simulink model "r23_512p_fft"  (R2026b)
settings: Solver=FixedStepDiscrete  StopTime=5e-5*(127-1)  FixedStep=5e-5
libraries: dspsrcs4 x8
(part 2 of 3)

== matlab function r23_512p_fft/FFT_TOP/calc_unit29/r2_unit ==
  data: si_cha input; so_cha output; so_chb output; si_chb input
function [so_cha, so_chb] = r2_unit(si_cha, si_chb)
%R2_UNIT Radix-2 butterfly.

DW = 15;
fm = fimath('RoundingMethod', 'Nearest', 'OverflowAction', 'Saturate', ...
    'ProductMode', 'FullPrecision', 'SumMode', 'FullPrecision');

so_cha = fi(zeros(1, 2), 1, DW, 0, fm);
so_chb = fi(zeros(1, 2), 1, DW, 0, fm);
so_cha(:) = si_cha + si_chb;
so_chb(:) = si_cha - si_chb;
end

== matlab function r23_512p_fft/FFT_TOP/calc_unit34/r2_unit ==
  data: si_cha input; so_cha output; so_chb output; si_chb input
function [so_cha, so_chb] = r2_unit(si_cha, si_chb)
%R2_UNIT Radix-2 butterfly.

DW = 16;
fm = fimath('RoundingMethod', 'Nearest', 'OverflowAction', 'Saturate', ...
    'ProductMode', 'FullPrecision', 'SumMode', 'FullPrecision');

so_cha = fi(zeros(1, 2), 1, DW, 0, fm);
so_chb = fi(zeros(1, 2), 1, DW, 0, fm);
so_cha(:) = si_cha + si_chb;
so_chb(:) = si_cha - si_chb;
end

== matlab function r23_512p_fft/FFT_TOP/calc_unit17/pwr_unit ==
  data: si_cha input; so_cha output; so_chb output; si_chb input
function [so_cha, so_chb] = pwr_unit(si_cha, si_chb)
%PWR_UNIT Twiddle multiply before the butterfly: W^0, W^128.

DW = 13;
fm = fimath('RoundingMethod', 'Nearest', 'OverflowAction', 'Saturate', ...
    'ProductMode', 'FullPrecision', 'SumMode', 'FullPrecision');

so_cha = mul_one(si_cha, DW, fm);
so_chb = mul_neg_j(si_chb, DW, fm);
end

function y = mul_one(x, DW, fm)
y = fi(zeros(1, 2), 1, DW, 0, fm);
y(:) = x;
end

function y = mul_neg_j(x, DW, fm)
y = fi(zeros(1, 2), 1, DW, 0, fm);
y(1) = x(2);
y(2) = -x(1);
end

== matlab function r23_512p_fft/FFT_TOP/calc_unit35/r2_unit ==
  data: si_cha input; so_cha output; so_chb output; si_chb input
function [so_cha, so_chb] = r2_unit(si_cha, si_chb)
%R2_UNIT Radix-2 butterfly.

DW = 16;
fm = fimath('RoundingMethod', 'Nearest', 'OverflowAction', 'Saturate', ...
    'ProductMode', 'FullPrecision', 'SumMode', 'FullPrecision');

so_cha = fi(zeros(1, 2), 1, DW, 0, fm);
so_chb = fi(zeros(1, 2), 1, DW, 0, fm);
so_cha(:) = si_cha + si_chb;
so_chb(:) = si_cha - si_chb;
end

== matlab function r23_512p_fft/FFT_TOP/calc_unit32/r2_unit ==
  data: si_cha input; so_cha output; so_chb output; si_chb input
function [so_cha, so_chb] = r2_unit(si_cha, si_chb)
%R2_UNIT Radix-2 butterfly.

DW = 16;
fm = fimath('RoundingMethod', 'Nearest', 'OverflowAction', 'Saturate', ...
    'ProductMode', 'FullPrecision', 'SumMode', 'FullPrecision');

so_cha = fi(zeros(1, 2), 1, DW, 0, fm);
so_chb = fi(zeros(1, 2), 1, DW, 0, fm);
so_cha(:) = si_cha + si_chb;
so_chb(:) = si_cha - si_chb;
end

== matlab function r23_512p_fft/FFT_TOP/calc_unit0/r2_unit ==
  data: si_cha input; so_cha output; so_chb output; si_chb input
function [so_cha, so_chb] = r2_unit(si_cha, si_chb)
%R2_UNIT Radix-2 butterfly.

DW = 12;
fm = fimath('RoundingMethod', 'Nearest', 'OverflowAction', 'Saturate', ...
    'ProductMode', 'FullPrecision', 'SumMode', 'FullPrecision');

so_cha = fi(zeros(1, 2), 1, DW, 0, fm);
so_chb = fi(zeros(1, 2), 1, DW, 0, fm);
so_cha(:) = si_cha + si_chb;
so_chb(:) = si_cha - si_chb;
end

== matlab function r23_512p_fft/FFT_TOP/calc_unit33/r2_unit ==
  data: si_cha input; so_cha output; so_chb output; si_chb input
function [so_cha, so_chb] = r2_unit(si_cha, si_chb)
%R2_UNIT Radix-2 butterfly.

DW = 16;
fm = fimath('RoundingMethod', 'Nearest', 'OverflowAction', 'Saturate', ...
    'ProductMode', 'FullPrecision', 'SumMode', 'FullPrecision');

so_cha = fi(zeros(1, 2), 1, DW, 0, fm);
so_chb = fi(zeros(1, 2), 1, DW, 0, fm);
so_cha(:) = si_cha + si_chb;
so_chb(:) = si_cha - si_chb;
end

== matlab function r23_512p_fft/FFT_TOP/comm_unit01/sw_unit ==
  data: si_cha input; so_cha output; so_chb output; si_chb input
function [so_cha, so_chb] = sw_unit(si_cha, si_chb)
%SW_UNIT Commutator switch, depth 32.

N  = 32;
CW = 5;
DW = 12;
fm = fimath('RoundingMethod', 'Nearest', 'OverflowAction', 'Saturate', ...
    'ProductMode', 'FullPrecision', 'SumMode', 'FullPrecision');
fc = fimath('RoundingMethod', 'Floor', 'OverflowAction', 'Wrap', ...
    'ProductMode', 'FullPrecision', 'SumMode', 'FullPrecision');

persistent cnt sel
if isempty(cnt)
    cnt = fi(N - 1, 0, CW, 0, fc);
end
if isempty(sel)
    sel = true;
end

if cnt == N - 1
    cnt(:) = 0;
else
    cnt(:) = cnt + 1;
end
if cnt == 0
    sel = ~sel;
end

so_cha = fi(zeros(1, 2), 1, DW, 0, fm);
so_chb = fi(zeros(1, 2), 1, DW, 0, fm);
if sel
    so_cha(:) = si_chb;
    so_chb(:) = si_cha;
else
    so_cha(:) = si_cha;
    so_chb(:) = si_chb;
end
end

== matlab function r23_512p_fft/FFT_TOP/comm_unit02/sw_unit ==
  data: si_cha input; so_cha output; so_chb output; si_chb input
function [so_cha, so_chb] = sw_unit(si_cha, si_chb)
%SW_UNIT Commutator switch, depth 32.

N  = 32;
CW = 5;
DW = 12;
fm = fimath('RoundingMethod', 'Nearest', 'OverflowAction', 'Saturate', ...
    'ProductMode', 'FullPrecision', 'SumMode', 'FullPrecision');
fc = fimath('RoundingMethod', 'Floor', 'OverflowAction', 'Wrap', ...
    'ProductMode', 'FullPrecision', 'SumMode', 'FullPrecision');

persistent cnt sel
if isempty(cnt)
    cnt = fi(N - 1, 0, CW, 0, fc);
end
if isempty(sel)
    sel = true;
end

if cnt == N - 1
    cnt(:) = 0;
else
    cnt(:) = cnt + 1;
end
if cnt == 0
    sel = ~sel;
end

so_cha = fi(zeros(1, 2), 1, DW, 0, fm);
so_chb = fi(zeros(1, 2), 1, DW, 0, fm);
if sel
    so_cha(:) = si_chb;
    so_chb(:) = si_cha;
else
    so_cha(:) = si_cha;
    so_chb(:) = si_chb;
end
end

== matlab function r23_512p_fft/FFT_TOP/calc_unit19/pwr_unit ==
  data: si_cha input; so_cha output; so_chb output; si_chb input
function [so_cha, so_chb] = pwr_unit(si_cha, si_chb)
%PWR_UNIT Twiddle multiply before the butterfly: W^0, W^128.

DW = 13;
fm = fimath('RoundingMethod', 'Nearest', 'OverflowAction', 'Saturate', ...
    'ProductMode', 'FullPrecision', 'SumMode', 'FullPrecision');

so_cha = mul_one(si_cha, DW, fm);
so_chb = mul_neg_j(si_chb, DW, fm);
end

function y = mul_one(x, DW, fm)
y = fi(zeros(1, 2), 1, DW, 0, fm);
y(:) = x;
end

function y = mul_neg_j(x, DW, fm)
y = fi(zeros(1, 2), 1, DW, 0, fm);
y(1) = x(2);
y(2) = -x(1);
end

== matlab function r23_512p_fft/FFT_TOP/comm_unit03/sw_unit ==
  data: si_cha input; so_cha output; so_chb output; si_chb input
function [so_cha, so_chb] = sw_unit(si_cha, si_chb)
%SW_UNIT Commutator switch, depth 32.

N  = 32;
CW = 5;
DW = 12;
fm = fimath('RoundingMethod', 'Nearest', 'OverflowAction', 'Saturate', ...
    'ProductMode', 'FullPrecision', 'SumMode', 'FullPrecision');
fc = fimath('RoundingMethod', 'Floor', 'OverflowAction', 'Wrap', ...
    'ProductMode', 'FullPrecision', 'SumMode', 'FullPrecision');

persistent cnt sel
if isempty(cnt)
    cnt = fi(N - 1, 0, CW, 0, fc);
end
if isempty(sel)
    sel = true;
end

if cnt == N - 1
    cnt(:) = 0;
else
    cnt(:) = cnt + 1;
end
if cnt == 0
    sel = ~sel;
end

so_cha = fi(zeros(1, 2), 1, DW, 0, fm);
so_chb = fi(zeros(1, 2), 1, DW, 0, fm);
if sel
    so_cha(:) = si_chb;
    so_chb(:) = si_cha;
else
    so_cha(:) = si_cha;
    so_chb(:) = si_chb;
end
end

== matlab function r23_512p_fft/FFT_TOP/comm_unit10/sw_unit ==
  data: si_cha input; so_cha output; so_chb output; si_chb input
function [so_cha, so_chb] = sw_unit(si_cha, si_chb)
%SW_UNIT Commutator switch, depth 16.

N  = 16;
CW = 4;
DW = 13;
fm = fimath('RoundingMethod', 'Nearest', 'OverflowAction', 'Saturate', ...
    'ProductMode', 'FullPrecision', 'SumMode', 'FullPrecision');
fc = fimath('RoundingMethod', 'Floor', 'OverflowAction', 'Wrap', ...
    'ProductMode', 'FullPrecision', 'SumMode', 'FullPrecision');

persistent cnt sel
if isempty(cnt)
    cnt = fi(N - 1, 0, CW, 0, fc);
end
if isempty(sel)
    sel = true;
end

if cnt == N - 1
    cnt(:) = 0;
else
    cnt(:) = cnt + 1;
end
if cnt == 0
    sel = ~sel;
end

so_cha = fi(zeros(1, 2), 1, DW, 0, fm);
so_chb = fi(zeros(1, 2), 1, DW, 0, fm);
if sel
    so_cha(:) = si_chb;
    so_chb(:) = si_cha;
else
    so_cha(:) = si_cha;
    so_chb(:) = si_chb;
end
end

== matlab function r23_512p_fft/FFT_TOP/comm_unit11/sw_unit ==
  data: si_cha input; so_cha output; so_chb output; si_chb input
function [so_cha, so_chb] = sw_unit(si_cha, si_chb)
%SW_UNIT Commutator switch, depth 16.

N  = 16;
CW = 4;
DW = 13;
fm = fimath('RoundingMethod', 'Nearest', 'OverflowAction', 'Saturate', ...
    'ProductMode', 'FullPrecision', 'SumMode', 'FullPrecision');
fc = fimath('RoundingMethod', 'Floor', 'OverflowAction', 'Wrap', ...
    'ProductMode', 'FullPrecision', 'SumMode', 'FullPrecision');

persistent cnt sel
if isempty(cnt)
    cnt = fi(N - 1, 0, CW, 0, fc);
end
if isempty(sel)
    sel = true;
end

if cnt == N - 1
    cnt(:) = 0;
else
    cnt(:) = cnt + 1;
end
if cnt == 0
    sel = ~sel;
end

so_cha = fi(zeros(1, 2), 1, DW, 0, fm);
so_chb = fi(zeros(1, 2), 1, DW, 0, fm);
if sel
    so_cha(:) = si_chb;
    so_chb(:) = si_cha;
else
    so_cha(:) = si_cha;
    so_chb(:) = si_chb;
end
end

== matlab function r23_512p_fft/FFT_TOP/calc_unit2/r2_unit ==
  data: si_cha input; so_cha output; so_chb output; si_chb input
function [so_cha, so_chb] = r2_unit(si_cha, si_chb)
%R2_UNIT Radix-2 butterfly.

DW = 12;
fm = fimath('RoundingMethod', 'Nearest', 'OverflowAction', 'Saturate', ...
    'ProductMode', 'FullPrecision', 'SumMode', 'FullPrecision');

so_cha = fi(zeros(1, 2), 1, DW, 0, fm);
so_chb = fi(zeros(1, 2), 1, DW, 0, fm);
so_cha(:) = si_cha + si_chb;
so_chb(:) = si_cha - si_chb;
end

== matlab function r23_512p_fft/FFT_TOP/calc_unit20/bwr_unit ==
  data: si_cha input; so_cha output; so_chb output; si_chb input
function [so_cha, so_chb] = bwr_unit(si_cha, si_chb)
%BWR_UNIT Twiddle multiply after the butterfly: W^(8k), W^(40k), k = 0..7.

DW = 15;
LEN = 8;
KW  = 3;
fm = fimath('RoundingMethod', 'Nearest', 'OverflowAction', 'Saturate', ...
    'ProductMode', 'FullPrecision', 'SumMode', 'FullPrecision');
fc = fimath('RoundingMethod', 'Floor', 'OverflowAction', 'Wrap', ...
    'ProductMode', 'FullPrecision', 'SumMode', 'FullPrecision');
ROM_A_RE = coder.const(twiddle((0:LEN-1).' * 8, 1, fm));
ROM_A_IM = coder.const(twiddle((0:LEN-1).' * 8, 2, fm));
ROM_B_RE = coder.const(twiddle((0:LEN-1).' * 40, 1, fm));
ROM_B_IM = coder.const(twiddle((0:LEN-1).' * 40, 2, fm));

persistent k
if isempty(k)
    k = fi(LEN - 1, 0, KW, 0, fc);
end
if k == LEN - 1
    k(:) = 0;
else
    k(:) = k + 1;
end

so_cha = cmul(si_cha, [ROM_A_RE(k + 1), ROM_A_IM(k + 1)], DW, fm);
so_chb = cmul(si_chb, [ROM_B_RE(k + 1), ROM_B_IM(k + 1)], DW, fm);
end

function y = cmul(x, w, DW, fm)
y = fi(zeros(1, 2), 1, DW, 0, fm);
y(1) = x(1)*w(1) - x(2)*w(2);
y(2) = x(2)*w(1) + x(1)*w(2);
end

function w = twiddle(k, part, fm)
if part == 1
    w = fi(cos(2*pi*k/512), 1, 10, 8, fm);
else
    w = fi(-sin(2*pi*k/512), 1, 10, 8, fm);
end
end

== matlab function r23_512p_fft/FFT_TOP/calc_unit20/pwr_unit ==
  data: si_cha input; so_cha output; so_chb output; si_chb input
function [so_cha, so_chb] = pwr_unit(si_cha, si_chb)
%PWR_UNIT Twiddle multiply before the butterfly: W^0, W^64.

DW = 14;
fm = fimath('RoundingMethod', 'Nearest', 'OverflowAction', 'Saturate', ...
    'ProductMode', 'FullPrecision', 'SumMode', 'FullPrecision');
W_B = coder.const([twiddle(64, 1, fm), twiddle(64, 2, fm)]);

so_cha = mul_one(si_cha, DW, fm);
so_chb = cmul(si_chb, W_B, DW, fm);
end

function y = mul_one(x, DW, fm)
y = fi(zeros(1, 2), 1, DW, 0, fm);
y(:) = x;
end

function y = cmul(x, w, DW, fm)
y = fi(zeros(1, 2), 1, DW, 0, fm);
y(1) = x(1)*w(1) - x(2)*w(2);
y(2) = x(2)*w(1) + x(1)*w(2);
end

function w = twiddle(k, part, fm)
if part == 1
    w = fi(cos(2*pi*k/512), 1, 10, 8, fm);
else
    w = fi(-sin(2*pi*k/512), 1, 10, 8, fm);
end
end

== matlab function r23_512p_fft/FFT_TOP/calc_unit1/bwr_unit ==
  data: si_cha input; so_cha output; so_chb output; si_chb input
function [so_cha, so_chb] = bwr_unit(si_cha, si_chb)
%BWR_UNIT Twiddle multiply after the butterfly: W^0, W^128.

DW = 12;
fm = fimath('RoundingMethod', 'Nearest', 'OverflowAction', 'Saturate', ...
    'ProductMode', 'FullPrecision', 'SumMode', 'FullPrecision');

so_cha = mul_one(si_cha, DW, fm);
so_chb = mul_neg_j(si_chb, DW, fm);
end

function y = mul_one(x, DW, fm)
y = fi(zeros(1, 2), 1, DW, 0, fm);
y(:) = x;
end

function y = mul_neg_j(x, DW, fm)
y = fi(zeros(1, 2), 1, DW, 0, fm);
y(1) = x(2);
y(2) = -x(1);
end

== matlab function r23_512p_fft/FFT_TOP/comm_unit12/sw_unit ==
  data: si_cha input; so_cha output; so_chb output; si_chb input
function [so_cha, so_chb] = sw_unit(si_cha, si_chb)
%SW_UNIT Commutator switch, depth 16.

N  = 16;
CW = 4;
DW = 13;
fm = fimath('RoundingMethod', 'Nearest', 'OverflowAction', 'Saturate', ...
    'ProductMode', 'FullPrecision', 'SumMode', 'FullPrecision');
fc = fimath('RoundingMethod', 'Floor', 'OverflowAction', 'Wrap', ...
    'ProductMode', 'FullPrecision', 'SumMode', 'FullPrecision');

persistent cnt sel
if isempty(cnt)
    cnt = fi(N - 1, 0, CW, 0, fc);
end
if isempty(sel)
    sel = true;
end

if cnt == N - 1
    cnt(:) = 0;
else
    cnt(:) = cnt + 1;
end
if cnt == 0
    sel = ~sel;
end

so_cha = fi(zeros(1, 2), 1, DW, 0, fm);
so_chb = fi(zeros(1, 2), 1, DW, 0, fm);
if sel
    so_cha(:) = si_chb;
    so_chb(:) = si_cha;
else
    so_cha(:) = si_cha;
    so_chb(:) = si_chb;
end
end

== matlab function r23_512p_fft/FFT_TOP/calc_unit21/bwr_unit ==
  data: si_cha input; so_cha output; so_chb output; si_chb input
function [so_cha, so_chb] = bwr_unit(si_cha, si_chb)
%BWR_UNIT Twiddle multiply after the butterfly: W^(24k), W^(56k), k = 0..7.

DW = 15;
LEN = 8;
KW  = 3;
fm = fimath('RoundingMethod', 'Nearest', 'OverflowAction', 'Saturate', ...
    'ProductMode', 'FullPrecision', 'SumMode', 'FullPrecision');
fc = fimath('RoundingMethod', 'Floor', 'OverflowAction', 'Wrap', ...
    'ProductMode', 'FullPrecision', 'SumMode', 'FullPrecision');
ROM_A_RE = coder.const(twiddle((0:LEN-1).' * 24, 1, fm));
ROM_A_IM = coder.const(twiddle((0:LEN-1).' * 24, 2, fm));
ROM_B_RE = coder.const(twiddle((0:LEN-1).' * 56, 1, fm));
ROM_B_IM = coder.const(twiddle((0:LEN-1).' * 56, 2, fm));

persistent k
if isempty(k)
    k = fi(LEN - 1, 0, KW, 0, fc);
end
if k == LEN - 1
    k(:) = 0;
else
    k(:) = k + 1;
end

so_cha = cmul(si_cha, [ROM_A_RE(k + 1), ROM_A_IM(k + 1)], DW, fm);
so_chb = cmul(si_chb, [ROM_B_RE(k + 1), ROM_B_IM(k + 1)], DW, fm);
end

function y = cmul(x, w, DW, fm)
y = fi(zeros(1, 2), 1, DW, 0, fm);
y(1) = x(1)*w(1) - x(2)*w(2);
y(2) = x(2)*w(1) + x(1)*w(2);
end

function w = twiddle(k, part, fm)
if part == 1
    w = fi(cos(2*pi*k/512), 1, 10, 8, fm);
else
    w = fi(-sin(2*pi*k/512), 1, 10, 8, fm);
end
end

== matlab function r23_512p_fft/FFT_TOP/calc_unit21/pwr_unit ==
  data: si_cha input; so_cha output; so_chb output; si_chb input
function [so_cha, so_chb] = pwr_unit(si_cha, si_chb)
%PWR_UNIT Twiddle multiply before the butterfly: W^0, W^192.

DW = 14;
fm = fimath('RoundingMethod', 'Nearest', 'OverflowAction', 'Saturate', ...
    'ProductMode', 'FullPrecision', 'SumMode', 'FullPrecision');
W_B = coder.const([twiddle(192, 1, fm), twiddle(192, 2, fm)]);

so_cha = mul_one(si_cha, DW, fm);
so_chb = cmul(si_chb, W_B, DW, fm);
end

function y = mul_one(x, DW, fm)
y = fi(zeros(1, 2), 1, DW, 0, fm);
y(:) = x;
end

function y = cmul(x, w, DW, fm)
y = fi(zeros(1, 2), 1, DW, 0, fm);
y(1) = x(1)*w(1) - x(2)*w(2);
y(2) = x(2)*w(1) + x(1)*w(2);
end

function w = twiddle(k, part, fm)
if part == 1
    w = fi(cos(2*pi*k/512), 1, 10, 8, fm);
else
    w = fi(-sin(2*pi*k/512), 1, 10, 8, fm);
end
end

== matlab function r23_512p_fft/FFT_TOP/comm_unit13/sw_unit ==
  data: si_cha input; so_cha output; so_chb output; si_chb input
function [so_cha, so_chb] = sw_unit(si_cha, si_chb)
%SW_UNIT Commutator switch, depth 16.

N  = 16;
CW = 4;
DW = 13;
fm = fimath('RoundingMethod', 'Nearest', 'OverflowAction', 'Saturate', ...
    'ProductMode', 'FullPrecision', 'SumMode', 'FullPrecision');
fc = fimath('RoundingMethod', 'Floor', 'OverflowAction', 'Wrap', ...
    'ProductMode', 'FullPrecision', 'SumMode', 'FullPrecision');

persistent cnt sel
if isempty(cnt)
    cnt = fi(N - 1, 0, CW, 0, fc);
end
if isempty(sel)
    sel = true;
end

if cnt == N - 1
    cnt(:) = 0;
else
    cnt(:) = cnt + 1;
end
if cnt == 0
    sel = ~sel;
end

so_cha = fi(zeros(1, 2), 1, DW, 0, fm);
so_chb = fi(zeros(1, 2), 1, DW, 0, fm);
if sel
    so_cha(:) = si_chb;
    so_chb(:) = si_cha;
else
    so_cha(:) = si_cha;
    so_chb(:) = si_chb;
end
end

== matlab function r23_512p_fft/FFT_TOP/calc_unit22/bwr_unit ==
  data: si_cha input; so_cha output; so_chb output; si_chb input
function [so_cha, so_chb] = bwr_unit(si_cha, si_chb)
%BWR_UNIT Twiddle multiply after the butterfly: W^0, W^(32k), k = 0..7.

DW = 15;
LEN = 8;
KW  = 3;
fm = fimath('RoundingMethod', 'Nearest', 'OverflowAction', 'Saturate', ...
    'ProductMode', 'FullPrecision', 'SumMode', 'FullPrecision');
fc = fimath('RoundingMethod', 'Floor', 'OverflowAction', 'Wrap', ...
    'ProductMode', 'FullPrecision', 'SumMode', 'FullPrecision');
ROM_B_RE = coder.const(twiddle((0:LEN-1).' * 32, 1, fm));
ROM_B_IM = coder.const(twiddle((0:LEN-1).' * 32, 2, fm));

persistent k
if isempty(k)
    k = fi(LEN - 1, 0, KW, 0, fc);
end
if k == LEN - 1
    k(:) = 0;
else
    k(:) = k + 1;
end

so_cha = mul_one(si_cha, DW, fm);
so_chb = cmul(si_chb, [ROM_B_RE(k + 1), ROM_B_IM(k + 1)], DW, fm);
end

function y = mul_one(x, DW, fm)
y = fi(zeros(1, 2), 1, DW, 0, fm);
y(:) = x;
end

function y = cmul(x, w, DW, fm)
y = fi(zeros(1, 2), 1, DW, 0, fm);
y(1) = x(1)*w(1) - x(2)*w(2);
y(2) = x(2)*w(1) + x(1)*w(2);
end

function w = twiddle(k, part, fm)
if part == 1
    w = fi(cos(2*pi*k/512), 1, 10, 8, fm);
else
    w = fi(-sin(2*pi*k/512), 1, 10, 8, fm);
end
end

== matlab function r23_512p_fft/FFT_TOP/comm_unit20/sw_unit ==
  data: si_cha input; so_cha output; so_chb output; si_chb input
function [so_cha, so_chb] = sw_unit(si_cha, si_chb)
%SW_UNIT Commutator switch, depth 8.

N  = 8;
CW = 3;
DW = 14;
fm = fimath('RoundingMethod', 'Nearest', 'OverflowAction', 'Saturate', ...
    'ProductMode', 'FullPrecision', 'SumMode', 'FullPrecision');
fc = fimath('RoundingMethod', 'Floor', 'OverflowAction', 'Wrap', ...
    'ProductMode', 'FullPrecision', 'SumMode', 'FullPrecision');

persistent cnt sel
if isempty(cnt)
    cnt = fi(N - 1, 0, CW, 0, fc);
end
if isempty(sel)
    sel = true;
end

if cnt == N - 1
    cnt(:) = 0;
else
    cnt(:) = cnt + 1;
end
if cnt == 0
    sel = ~sel;
end

so_cha = fi(zeros(1, 2), 1, DW, 0, fm);
so_chb = fi(zeros(1, 2), 1, DW, 0, fm);
if sel
    so_cha(:) = si_chb;
    so_chb(:) = si_cha;
else
    so_cha(:) = si_cha;
    so_chb(:) = si_chb;
end
end

== matlab function r23_512p_fft/FFT_TOP/comm_unit21/sw_unit ==
  data: si_cha input; so_cha output; so_chb output; si_chb input
function [so_cha, so_chb] = sw_unit(si_cha, si_chb)
%SW_UNIT Commutator switch, depth 8.

N  = 8;
CW = 3;
DW = 14;
fm = fimath('RoundingMethod', 'Nearest', 'OverflowAction', 'Saturate', ...
    'ProductMode', 'FullPrecision', 'SumMode', 'FullPrecision');
fc = fimath('RoundingMethod', 'Floor', 'OverflowAction', 'Wrap', ...
    'ProductMode', 'FullPrecision', 'SumMode', 'FullPrecision');

persistent cnt sel
if isempty(cnt)
    cnt = fi(N - 1, 0, CW, 0, fc);
end
if isempty(sel)
    sel = true;
end

if cnt == N - 1
    cnt(:) = 0;
else
    cnt(:) = cnt + 1;
end
if cnt == 0
    sel = ~sel;
end

so_cha = fi(zeros(1, 2), 1, DW, 0, fm);
so_chb = fi(zeros(1, 2), 1, DW, 0, fm);
if sel
    so_cha(:) = si_chb;
    so_chb(:) = si_cha;
else
    so_cha(:) = si_cha;
    so_chb(:) = si_chb;
end
end

== matlab function r23_512p_fft/FFT_TOP/calc_unit23/bwr_unit ==
  data: si_cha input; so_cha output; so_chb output; si_chb input
function [so_cha, so_chb] = bwr_unit(si_cha, si_chb)
%BWR_UNIT Twiddle multiply after the butterfly: W^(16k), W^(48k), k = 0..7.

DW = 15;
LEN = 8;
KW  = 3;
fm = fimath('RoundingMethod', 'Nearest', 'OverflowAction', 'Saturate', ...
    'ProductMode', 'FullPrecision', 'SumMode', 'FullPrecision');
fc = fimath('RoundingMethod', 'Floor', 'OverflowAction', 'Wrap', ...
    'ProductMode', 'FullPrecision', 'SumMode', 'FullPrecision');
ROM_A_RE = coder.const(twiddle((0:LEN-1).' * 16, 1, fm));
ROM_A_IM = coder.const(twiddle((0:LEN-1).' * 16, 2, fm));
ROM_B_RE = coder.const(twiddle((0:LEN-1).' * 48, 1, fm));
ROM_B_IM = coder.const(twiddle((0:LEN-1).' * 48, 2, fm));

persistent k
if isempty(k)
    k = fi(LEN - 1, 0, KW, 0, fc);
end
if k == LEN - 1
    k(:) = 0;
else
    k(:) = k + 1;
end

so_cha = cmul(si_cha, [ROM_A_RE(k + 1), ROM_A_IM(k + 1)], DW, fm);
so_chb = cmul(si_chb, [ROM_B_RE(k + 1), ROM_B_IM(k + 1)], DW, fm);
end

function y = cmul(x, w, DW, fm)
y = fi(zeros(1, 2), 1, DW, 0, fm);
y(1) = x(1)*w(1) - x(2)*w(2);
y(2) = x(2)*w(1) + x(1)*w(2);
end

function w = twiddle(k, part, fm)
if part == 1
    w = fi(cos(2*pi*k/512), 1, 10, 8, fm);
else
    w = fi(-sin(2*pi*k/512), 1, 10, 8, fm);
end
end

== matlab function r23_512p_fft/FFT_TOP/calc_unit23/pwr_unit ==
  data: si_cha input; so_cha output; so_chb output; si_chb input
function [so_cha, so_chb] = pwr_unit(si_cha, si_chb)
%PWR_UNIT Twiddle multiply before the butterfly: W^0, W^128.

DW = 14;
fm = fimath('RoundingMethod', 'Nearest', 'OverflowAction', 'Saturate', ...
    'ProductMode', 'FullPrecision', 'SumMode', 'FullPrecision');

so_cha = mul_one(si_cha, DW, fm);
so_chb = mul_neg_j(si_chb, DW, fm);
end

function y = mul_one(x, DW, fm)
y = fi(zeros(1, 2), 1, DW, 0, fm);
y(:) = x;
end

function y = mul_neg_j(x, DW, fm)
y = fi(zeros(1, 2), 1, DW, 0, fm);
y(1) = x(2);
y(2) = -x(1);
end

== matlab function r23_512p_fft/FFT_TOP/comm_unit22/sw_unit ==
  data: si_cha input; so_cha output; so_chb output; si_chb input
function [so_cha, so_chb] = sw_unit(si_cha, si_chb)
%SW_UNIT Commutator switch, depth 8.

N  = 8;
CW = 3;
DW = 14;
fm = fimath('RoundingMethod', 'Nearest', 'OverflowAction', 'Saturate', ...
    'ProductMode', 'FullPrecision', 'SumMode', 'FullPrecision');
fc = fimath('RoundingMethod', 'Floor', 'OverflowAction', 'Wrap', ...
    'ProductMode', 'FullPrecision', 'SumMode', 'FullPrecision');

persistent cnt sel
if isempty(cnt)
    cnt = fi(N - 1, 0, CW, 0, fc);
end
if isempty(sel)
    sel = true;
end

if cnt == N - 1
    cnt(:) = 0;
else
    cnt(:) = cnt + 1;
end
if cnt == 0
    sel = ~sel;
end

so_cha = fi(zeros(1, 2), 1, DW, 0, fm);
so_chb = fi(zeros(1, 2), 1, DW, 0, fm);
if sel
    so_cha(:) = si_chb;
    so_chb(:) = si_cha;
else
    so_cha(:) = si_cha;
    so_chb(:) = si_chb;
end
end

== matlab function r23_512p_fft/FFT_TOP/calc_unit14/r2_unit ==
  data: si_cha input; so_cha output; so_chb output; si_chb input
function [so_cha, so_chb] = r2_unit(si_cha, si_chb)
%R2_UNIT Radix-2 butterfly.

DW = 13;
fm = fimath('RoundingMethod', 'Nearest', 'OverflowAction', 'Saturate', ...
    'ProductMode', 'FullPrecision', 'SumMode', 'FullPrecision');

so_cha = fi(zeros(1, 2), 1, DW, 0, fm);
so_chb = fi(zeros(1, 2), 1, DW, 0, fm);
so_cha(:) = si_cha + si_chb;
so_chb(:) = si_cha - si_chb;
end

== matlab function r23_512p_fft/FFT_TOP/comm_unit23/sw_unit ==
  data: si_cha input; so_cha output; so_chb output; si_chb input
function [so_cha, so_chb] = sw_unit(si_cha, si_chb)
%SW_UNIT Commutator switch, depth 8.

N  = 8;
CW = 3;
DW = 14;
fm = fimath('RoundingMethod', 'Nearest', 'OverflowAction', 'Saturate', ...
    'ProductMode', 'FullPrecision', 'SumMode', 'FullPrecision');
fc = fimath('RoundingMethod', 'Floor', 'OverflowAction', 'Wrap', ...
    'ProductMode', 'FullPrecision', 'SumMode', 'FullPrecision');

persistent cnt sel
if isempty(cnt)
    cnt = fi(N - 1, 0, CW, 0, fc);
end
if isempty(sel)
    sel = true;
end

if cnt == N - 1
    cnt(:) = 0;
else
    cnt(:) = cnt + 1;
end
if cnt == 0
    sel = ~sel;
end

so_cha = fi(zeros(1, 2), 1, DW, 0, fm);
so_chb = fi(zeros(1, 2), 1, DW, 0, fm);
if sel
    so_cha(:) = si_chb;
    so_chb(:) = si_cha;
else
    so_cha(:) = si_cha;
    so_chb(:) = si_chb;
end
end

== matlab function r23_512p_fft/FFT_TOP/comm_unit30/sw_unit ==
  data: si_cha input; so_cha output; so_chb output; si_chb input
function [so_cha, so_chb] = sw_unit(si_cha, si_chb)
%SW_UNIT Commutator switch, depth 4.

N  = 4;
CW = 2;
DW = 13;
fm = fimath('RoundingMethod', 'Nearest', 'OverflowAction', 'Saturate', ...
    'ProductMode', 'FullPrecision', 'SumMode', 'FullPrecision');
fc = fimath('RoundingMethod', 'Floor', 'OverflowAction', 'Wrap', ...
    'ProductMode', 'FullPrecision', 'SumMode', 'FullPrecision');

persistent cnt sel
if isempty(cnt)
    cnt = fi(N - 1, 0, CW, 0, fc);
end
if isempty(sel)
    sel = true;
end

if cnt == N - 1
    cnt(:) = 0;
else
    cnt(:) = cnt + 1;
end
if cnt == 0
    sel = ~sel;
end

so_cha = fi(zeros(1, 2), 1, DW, 0, fm);
so_chb = fi(zeros(1, 2), 1, DW, 0, fm);
if sel
    so_cha(:) = si_chb;
    so_chb(:) = si_cha;
else
    so_cha(:) = si_cha;
    so_chb(:) = si_chb;
end
end

== matlab function r23_512p_fft/FFT_TOP/comm_unit31/sw_unit ==
  data: si_cha input; so_cha output; so_chb output; si_chb input
function [so_cha, so_chb] = sw_unit(si_cha, si_chb)
%SW_UNIT Commutator switch, depth 4.

N  = 4;
CW = 2;
DW = 13;
fm = fimath('RoundingMethod', 'Nearest', 'OverflowAction', 'Saturate', ...
    'ProductMode', 'FullPrecision', 'SumMode', 'FullPrecision');
fc = fimath('RoundingMethod', 'Floor', 'OverflowAction', 'Wrap', ...
    'ProductMode', 'FullPrecision', 'SumMode', 'FullPrecision');

persistent cnt sel
if isempty(cnt)
    cnt = fi(N - 1, 0, CW, 0, fc);
end
if isempty(sel)
    sel = true;
end

if cnt == N - 1
    cnt(:) = 0;
else
    cnt(:) = cnt + 1;
end
if cnt == 0
    sel = ~sel;
end

so_cha = fi(zeros(1, 2), 1, DW, 0, fm);
so_chb = fi(zeros(1, 2), 1, DW, 0, fm);
if sel
    so_cha(:) = si_chb;
    so_chb(:) = si_cha;
else
    so_cha(:) = si_cha;
    so_chb(:) = si_chb;
end
end

== matlab function r23_512p_fft/FFT_TOP/comm_unit32/sw_unit ==
  data: si_cha input; so_cha output; so_chb output; si_chb input
function [so_cha, so_chb] = sw_unit(si_cha, si_chb)
%SW_UNIT Commutator switch, depth 4.

N  = 4;
CW = 2;
DW = 13;
fm = fimath('RoundingMethod', 'Nearest', 'OverflowAction', 'Saturate', ...
    'ProductMode', 'FullPrecision', 'SumMode', 'FullPrecision');
fc = fimath('RoundingMethod', 'Floor', 'OverflowAction', 'Wrap', ...
    'ProductMode', 'FullPrecision', 'SumMode', 'FullPrecision');

persistent cnt sel
if isempty(cnt)
    cnt = fi(N - 1, 0, CW, 0, fc);
end
if isempty(sel)
    sel = true;
end

if cnt == N - 1
    cnt(:) = 0;
else
    cnt(:) = cnt + 1;
end
if cnt == 0
    sel = ~sel;
end

so_cha = fi(zeros(1, 2), 1, DW, 0, fm);
so_chb = fi(zeros(1, 2), 1, DW, 0, fm);
if sel
    so_cha(:) = si_chb;
    so_chb(:) = si_cha;
else
    so_cha(:) = si_cha;
    so_chb(:) = si_chb;
end
end

== matlab function r23_512p_fft/FFT_TOP/comm_unit33/sw_unit ==
  data: si_cha input; so_cha output; so_chb output; si_chb input
function [so_cha, so_chb] = sw_unit(si_cha, si_chb)
%SW_UNIT Commutator switch, depth 4.

N  = 4;
CW = 2;
DW = 13;
fm = fimath('RoundingMethod', 'Nearest', 'OverflowAction', 'Saturate', ...
    'ProductMode', 'FullPrecision', 'SumMode', 'FullPrecision');
fc = fimath('RoundingMethod', 'Floor', 'OverflowAction', 'Wrap', ...
    'ProductMode', 'FullPrecision', 'SumMode', 'FullPrecision');

persistent cnt sel
if isempty(cnt)
    cnt = fi(N - 1, 0, CW, 0, fc);
end
if isempty(sel)
    sel = true;
end

if cnt == N - 1
    cnt(:) = 0;
else
    cnt(:) = cnt + 1;
end
if cnt == 0
    sel = ~sel;
end

so_cha = fi(zeros(1, 2), 1, DW, 0, fm);
so_chb = fi(zeros(1, 2), 1, DW, 0, fm);
if sel
    so_cha(:) = si_chb;
    so_chb(:) = si_cha;
else
    so_cha(:) = si_cha;
    so_chb(:) = si_chb;
end
end

== matlab function r23_512p_fft/FFT_TOP/comm_unit40/sw_unit ==
  data: si_cha input; so_cha output; so_chb output; si_chb input
function [so_cha, so_chb] = sw_unit(si_cha, si_chb)
%SW_UNIT Commutator switch, depth 2.

N  = 2;
CW = 1;
DW = 14;
fm = fimath('RoundingMethod', 'Nearest', 'OverflowAction', 'Saturate', ...
    'ProductMode', 'FullPrecision', 'SumMode', 'FullPrecision');
fc = fimath('RoundingMethod', 'Floor', 'OverflowAction', 'Wrap', ...
    'ProductMode', 'FullPrecision', 'SumMode', 'FullPrecision');

persistent cnt sel
if isempty(cnt)
    cnt = fi(N - 1, 0, CW, 0, fc);
end
if isempty(sel)
    sel = true;
end

if cnt == N - 1
    cnt(:) = 0;
else
    cnt(:) = cnt + 1;
end
if cnt == 0
    sel = ~sel;
end

so_cha = fi(zeros(1, 2), 1, DW, 0, fm);
so_chb = fi(zeros(1, 2), 1, DW, 0, fm);
if sel
    so_cha(:) = si_chb;
    so_chb(:) = si_cha;
else
    so_cha(:) = si_cha;
    so_chb(:) = si_chb;
end
end

== matlab function r23_512p_fft/FFT_TOP/comm_unit41/sw_unit ==
  data: si_cha input; so_cha output; so_chb output; si_chb input
function [so_cha, so_chb] = sw_unit(si_cha, si_chb)
%SW_UNIT Commutator switch, depth 2.

N  = 2;
CW = 1;
DW = 14;
fm = fimath('RoundingMethod', 'Nearest', 'OverflowAction', 'Saturate', ...
    'ProductMode', 'FullPrecision', 'SumMode', 'FullPrecision');
fc = fimath('RoundingMethod', 'Floor', 'OverflowAction', 'Wrap', ...
    'ProductMode', 'FullPrecision', 'SumMode', 'FullPrecision');

persistent cnt sel
if isempty(cnt)
    cnt = fi(N - 1, 0, CW, 0, fc);
end
if isempty(sel)
    sel = true;
end

if cnt == N - 1
    cnt(:) = 0;
else
    cnt(:) = cnt + 1;
end
if cnt == 0
    sel = ~sel;
end

so_cha = fi(zeros(1, 2), 1, DW, 0, fm);
so_chb = fi(zeros(1, 2), 1, DW, 0, fm);
if sel
    so_cha(:) = si_chb;
    so_chb(:) = si_cha;
else
    so_cha(:) = si_cha;
    so_chb(:) = si_chb;
end
end

== matlab function r23_512p_fft/FFT_TOP/comm_unit42/sw_unit ==
  data: si_cha input; so_cha output; so_chb output; si_chb input
function [so_cha, so_chb] = sw_unit(si_cha, si_chb)
%SW_UNIT Commutator switch, depth 2.

N  = 2;
CW = 1;
DW = 14;
fm = fimath('RoundingMethod', 'Nearest', 'OverflowAction', 'Saturate', ...
    'ProductMode', 'FullPrecision', 'SumMode', 'FullPrecision');
fc = fimath('RoundingMethod', 'Floor', 'OverflowAction', 'Wrap', ...
    'ProductMode', 'FullPrecision', 'SumMode', 'FullPrecision');

persistent cnt sel
if isempty(cnt)
    cnt = fi(N - 1, 0, CW, 0, fc);
end
if isempty(sel)
    sel = true;
end

if cnt == N - 1
    cnt(:) = 0;
else
    cnt(:) = cnt + 1;
end
if cnt == 0
    sel = ~sel;
end

so_cha = fi(zeros(1, 2), 1, DW, 0, fm);
so_chb = fi(zeros(1, 2), 1, DW, 0, fm);
if sel
    so_cha(:) = si_chb;
    so_chb(:) = si_cha;
else
    so_cha(:) = si_cha;
    so_chb(:) = si_chb;
end
end

== matlab function r23_512p_fft/FFT_TOP/comm_unit43/sw_unit ==
  data: si_cha input; so_cha output; so_chb output; si_chb input
function [so_cha, so_chb] = sw_unit(si_cha, si_chb)
%SW_UNIT Commutator switch, depth 2.

N  = 2;
CW = 1;
DW = 14;
fm = fimath('RoundingMethod', 'Nearest', 'OverflowAction', 'Saturate', ...
    'ProductMode', 'FullPrecision', 'SumMode', 'FullPrecision');
fc = fimath('RoundingMethod', 'Floor', 'OverflowAction', 'Wrap', ...
    'ProductMode', 'FullPrecision', 'SumMode', 'FullPrecision');

persistent cnt sel
if isempty(cnt)
    cnt = fi(N - 1, 0, CW, 0, fc);
end
if isempty(sel)
    sel = true;
end

if cnt == N - 1
    cnt(:) = 0;
else
    cnt(:) = cnt + 1;
end
if cnt == 0
    sel = ~sel;
end

so_cha = fi(zeros(1, 2), 1, DW, 0, fm);
so_chb = fi(zeros(1, 2), 1, DW, 0, fm);
if sel
    so_cha(:) = si_chb;
    so_chb(:) = si_cha;
else
    so_cha(:) = si_cha;
    so_chb(:) = si_chb;
end
end

== matlab function r23_512p_fft/FFT_TOP/comm_unit50/sw_unit ==
  data: si_cha input; so_cha output; so_chb output; si_chb input
function [so_cha, so_chb] = sw_unit(si_cha, si_chb)
%SW_UNIT Commutator switch, depth 1.

DW = 15;
fm = fimath('RoundingMethod', 'Nearest', 'OverflowAction', 'Saturate', ...
    'ProductMode', 'FullPrecision', 'SumMode', 'FullPrecision');

persistent sel
if isempty(sel)
    sel = true;
end
sel = ~sel;

so_cha = fi(zeros(1, 2), 1, DW, 0, fm);
so_chb = fi(zeros(1, 2), 1, DW, 0, fm);
if sel
    so_cha(:) = si_chb;
    so_chb(:) = si_cha;
else
    so_cha(:) = si_cha;
    so_chb(:) = si_chb;
end
end

== matlab function r23_512p_fft/FFT_TOP/calc_unit1/r2_unit ==
  data: si_cha input; so_cha output; so_chb output; si_chb input
function [so_cha, so_chb] = r2_unit(si_cha, si_chb)
%R2_UNIT Radix-2 butterfly.

DW = 12;
fm = fimath('RoundingMethod', 'Nearest', 'OverflowAction', 'Saturate', ...
    'ProductMode', 'FullPrecision', 'SumMode', 'FullPrecision');

so_cha = fi(zeros(1, 2), 1, DW, 0, fm);
so_chb = fi(zeros(1, 2), 1, DW, 0, fm);
so_cha(:) = si_cha + si_chb;
so_chb(:) = si_cha - si_chb;
end

== matlab function r23_512p_fft/FFT_TOP/comm_unit51/sw_unit ==
  data: si_cha input; so_cha output; so_chb output; si_chb input
function [so_cha, so_chb] = sw_unit(si_cha, si_chb)
%SW_UNIT Commutator switch, depth 1.

DW = 15;
fm = fimath('RoundingMethod', 'Nearest', 'OverflowAction', 'Saturate', ...
    'ProductMode', 'FullPrecision', 'SumMode', 'FullPrecision');

persistent sel
if isempty(sel)
    sel = true;
end
sel = ~sel;

so_cha = fi(zeros(1, 2), 1, DW, 0, fm);
so_chb = fi(zeros(1, 2), 1, DW, 0, fm);
if sel
    so_cha(:) = si_chb;
    so_chb(:) = si_cha;
else
    so_cha(:) = si_cha;
    so_chb(:) = si_chb;
end
end

== matlab function r23_512p_fft/FFT_TOP/comm_unit52/sw_unit ==
  data: si_cha input; so_cha output; so_chb output; si_chb input
function [so_cha, so_chb] = sw_unit(si_cha, si_chb)
%SW_UNIT Commutator switch, depth 1.

DW = 15;
fm = fimath('RoundingMethod', 'Nearest', 'OverflowAction', 'Saturate', ...
    'ProductMode', 'FullPrecision', 'SumMode', 'FullPrecision');

persistent sel
if isempty(sel)
    sel = true;
end
sel = ~sel;

so_cha = fi(zeros(1, 2), 1, DW, 0, fm);
so_chb = fi(zeros(1, 2), 1, DW, 0, fm);
if sel
    so_cha(:) = si_chb;
    so_chb(:) = si_cha;
else
    so_cha(:) = si_cha;
    so_chb(:) = si_chb;
end
end

== matlab function r23_512p_fft/FFT_TOP/comm_unit53/sw_unit ==
  data: si_cha input; so_cha output; so_chb output; si_chb input
function [so_cha, so_chb] = sw_unit(si_cha, si_chb)
%SW_UNIT Commutator switch, depth 1.

DW = 15;
fm = fimath('RoundingMethod', 'Nearest', 'OverflowAction', 'Saturate', ...
    'ProductMode', 'FullPrecision', 'SumMode', 'FullPrecision');

persistent sel
if isempty(sel)
    sel = true;
end
sel = ~sel;

so_cha = fi(zeros(1, 2), 1, DW, 0, fm);
so_chb = fi(zeros(1, 2), 1, DW, 0, fm);
if sel
    so_cha(:) = si_chb;
    so_chb(:) = si_cha;
else
    so_cha(:) = si_cha;
    so_chb(:) = si_chb;
end
end

== matlab function r23_512p_fft/FFT_TOP/calc_unit29/pwr_unit ==
  data: si_cha input; so_cha output; so_chb output; si_chb input
function [so_cha, so_chb] = pwr_unit(si_cha, si_chb)
%PWR_UNIT Twiddle multiply before the butterfly: W^0, W^128.

DW = 14;
fm = fimath('RoundingMethod', 'Nearest', 'OverflowAction', 'Saturate', ...
    'ProductMode', 'FullPrecision', 'SumMode', 'FullPrecision');

so_cha = mul_one(si_cha, DW, fm);
so_chb = mul_neg_j(si_chb, DW, fm);
end

function y = mul_one(x, DW, fm)
y = fi(zeros(1, 2), 1, DW, 0, fm);
y(:) = x;
end

function y = mul_neg_j(x, DW, fm)
y = fi(zeros(1, 2), 1, DW, 0, fm);
y(1) = x(2);
y(2) = -x(1);
end

== matlab function r23_512p_fft/FFT_TOP/calc_unit3/bwr_unit ==
  data: si_cha input; so_cha output; so_chb output; si_chb input
function [so_cha, so_chb] = bwr_unit(si_cha, si_chb)
%BWR_UNIT Twiddle multiply after the butterfly: W^0, W^128.

DW = 12;
fm = fimath('RoundingMethod', 'Nearest', 'OverflowAction', 'Saturate', ...
    'ProductMode', 'FullPrecision', 'SumMode', 'FullPrecision');

so_cha = mul_one(si_cha, DW, fm);
so_chb = mul_neg_j(si_chb, DW, fm);
end

function y = mul_one(x, DW, fm)
y = fi(zeros(1, 2), 1, DW, 0, fm);
y(:) = x;
end

function y = mul_neg_j(x, DW, fm)
y = fi(zeros(1, 2), 1, DW, 0, fm);
y(1) = x(2);
y(2) = -x(1);
end

== matlab function r23_512p_fft/FFT_TOP/calc_unit3/r2_unit ==
  data: si_cha input; so_cha output; so_chb output; si_chb input
function [so_cha, so_chb] = r2_unit(si_cha, si_chb)
%R2_UNIT Radix-2 butterfly.

DW = 12;
fm = fimath('RoundingMethod', 'Nearest', 'OverflowAction', 'Saturate', ...
    'ProductMode', 'FullPrecision', 'SumMode', 'FullPrecision');

so_cha = fi(zeros(1, 2), 1, DW, 0, fm);
so_chb = fi(zeros(1, 2), 1, DW, 0, fm);
so_cha(:) = si_cha + si_chb;
so_chb(:) = si_cha - si_chb;
end

== matlab function r23_512p_fft/FFT_TOP/calc_unit31/pwr_unit ==
  data: si_cha input; so_cha output; so_chb output; si_chb input
function [so_cha, so_chb] = pwr_unit(si_cha, si_chb)
%PWR_UNIT Twiddle multiply before the butterfly: W^0, W^128.

DW = 14;
fm = fimath('RoundingMethod', 'Nearest', 'OverflowAction', 'Saturate', ...
    'ProductMode', 'FullPrecision', 'SumMode', 'FullPrecision');

so_cha = mul_one(si_cha, DW, fm);
so_chb = mul_neg_j(si_chb, DW, fm);
end

function y = mul_one(x, DW, fm)
y = fi(zeros(1, 2), 1, DW, 0, fm);
y(:) = x;
end

function y = mul_neg_j(x, DW, fm)
y = fi(zeros(1, 2), 1, DW, 0, fm);
y(1) = x(2);
y(2) = -x(1);
end

== matlab function r23_512p_fft/FFT_TOP/calc_unit32/pwr_unit ==
  data: si_cha input; so_cha output; so_chb output; si_chb input
function [so_cha, so_chb] = pwr_unit(si_cha, si_chb)
%PWR_UNIT Twiddle multiply before the butterfly: W^0, W^64.

DW = 15;
fm = fimath('RoundingMethod', 'Nearest', 'OverflowAction', 'Saturate', ...
    'ProductMode', 'FullPrecision', 'SumMode', 'FullPrecision');
W_B = coder.const([twiddle(64, 1, fm), twiddle(64, 2, fm)]);

so_cha = mul_one(si_cha, DW, fm);
so_chb = cmul(si_chb, W_B, DW, fm);
end

function y = mul_one(x, DW, fm)
y = fi(zeros(1, 2), 1, DW, 0, fm);
y(:) = x;
end

function y = cmul(x, w, DW, fm)
y = fi(zeros(1, 2), 1, DW, 0, fm);
y(1) = x(1)*w(1) - x(2)*w(2);
y(2) = x(2)*w(1) + x(1)*w(2);
end

function w = twiddle(k, part, fm)
if part == 1
    w = fi(cos(2*pi*k/512), 1, 10, 8, fm);
else
    w = fi(-sin(2*pi*k/512), 1, 10, 8, fm);
end
end

== matlab function r23_512p_fft/FFT_TOP/calc_unit33/pwr_unit ==
  data: si_cha input; so_cha output; so_chb output; si_chb input
function [so_cha, so_chb] = pwr_unit(si_cha, si_chb)
%PWR_UNIT Twiddle multiply before the butterfly: W^0, W^192.

DW = 15;
fm = fimath('RoundingMethod', 'Nearest', 'OverflowAction', 'Saturate', ...
    'ProductMode', 'FullPrecision', 'SumMode', 'FullPrecision');
W_B = coder.const([twiddle(192, 1, fm), twiddle(192, 2, fm)]);

so_cha = mul_one(si_cha, DW, fm);
so_chb = cmul(si_chb, W_B, DW, fm);
end

function y = mul_one(x, DW, fm)
y = fi(zeros(1, 2), 1, DW, 0, fm);
y(:) = x;
end

function y = cmul(x, w, DW, fm)
y = fi(zeros(1, 2), 1, DW, 0, fm);
y(1) = x(1)*w(1) - x(2)*w(2);
y(2) = x(2)*w(1) + x(1)*w(2);
end

function w = twiddle(k, part, fm)
if part == 1
    w = fi(cos(2*pi*k/512), 1, 10, 8, fm);
else
    w = fi(-sin(2*pi*k/512), 1, 10, 8, fm);
end
end

== matlab function r23_512p_fft/FFT_TOP/calc_unit35/pwr_unit ==
  data: si_cha input; so_cha output; so_chb output; si_chb input
function [so_cha, so_chb] = pwr_unit(si_cha, si_chb)
%PWR_UNIT Twiddle multiply before the butterfly: W^0, W^128.

DW = 15;
fm = fimath('RoundingMethod', 'Nearest', 'OverflowAction', 'Saturate', ...
    'ProductMode', 'FullPrecision', 'SumMode', 'FullPrecision');

so_cha = mul_one(si_cha, DW, fm);
so_chb = mul_neg_j(si_chb, DW, fm);
end

function y = mul_one(x, DW, fm)
y = fi(zeros(1, 2), 1, DW, 0, fm);
y(:) = x;
end

function y = mul_neg_j(x, DW, fm)
y = fi(zeros(1, 2), 1, DW, 0, fm);
y(1) = x(2);
y(2) = -x(1);
end

== matlab function r23_512p_fft/FFT_TOP/calc_unit10/bwr_unit ==
  data: si_cha input; so_cha output; so_chb output; si_chb input
function [so_cha, so_chb] = bwr_unit(si_cha, si_chb)
%BWR_UNIT Twiddle multiply after the butterfly: W^(1k), W^(5k), k = 0..63.

DW = 14;
LEN = 64;
KW  = 6;
fm = fimath('RoundingMethod', 'Nearest', 'OverflowAction', 'Saturate', ...
    'ProductMode', 'FullPrecision', 'SumMode', 'FullPrecision');
fc = fimath('RoundingMethod', 'Floor', 'OverflowAction', 'Wrap', ...
    'ProductMode', 'FullPrecision', 'SumMode', 'FullPrecision');
ROM_A_RE = coder.const(twiddle((0:LEN-1).' * 1, 1, fm));
ROM_A_IM = coder.const(twiddle((0:LEN-1).' * 1, 2, fm));
ROM_B_RE = coder.const(twiddle((0:LEN-1).' * 5, 1, fm));
ROM_B_IM = coder.const(twiddle((0:LEN-1).' * 5, 2, fm));

persistent k
if isempty(k)
    k = fi(LEN - 1, 0, KW, 0, fc);
end
if k == LEN - 1
    k(:) = 0;
else
    k(:) = k + 1;
end

so_cha = cmul(si_cha, [ROM_A_RE(k + 1), ROM_A_IM(k + 1)], DW, fm);
so_chb = cmul(si_chb, [ROM_B_RE(k + 1), ROM_B_IM(k + 1)], DW, fm);
end

function y = cmul(x, w, DW, fm)
y = fi(zeros(1, 2), 1, DW, 0, fm);
y(1) = x(1)*w(1) - x(2)*w(2);
y(2) = x(2)*w(1) + x(1)*w(2);
end

function w = twiddle(k, part, fm)
if part == 1
    w = fi(cos(2*pi*k/512), 1, 10, 8, fm);
else
    w = fi(-sin(2*pi*k/512), 1, 10, 8, fm);
end
end

== matlab function r23_512p_fft/FFT_TOP/calc_unit4/r2_unit ==
  data: si_cha input; so_cha output; so_chb output; si_chb input
function [so_cha, so_chb] = r2_unit(si_cha, si_chb)
%R2_UNIT Radix-2 butterfly.

DW = 13;
fm = fimath('RoundingMethod', 'Nearest', 'OverflowAction', 'Saturate', ...
    'ProductMode', 'FullPrecision', 'SumMode', 'FullPrecision');

so_cha = fi(zeros(1, 2), 1, DW, 0, fm);
so_chb = fi(zeros(1, 2), 1, DW, 0, fm);
so_cha(:) = si_cha + si_chb;
so_chb(:) = si_cha - si_chb;
end

== matlab function r23_512p_fft/FFT_TOP/calc_unit5/r2_unit ==
  data: si_cha input; so_cha output; so_chb output; si_chb input
function [so_cha, so_chb] = r2_unit(si_cha, si_chb)
%R2_UNIT Radix-2 butterfly.

DW = 13;
fm = fimath('RoundingMethod', 'Nearest', 'OverflowAction', 'Saturate', ...
    'ProductMode', 'FullPrecision', 'SumMode', 'FullPrecision');

so_cha = fi(zeros(1, 2), 1, DW, 0, fm);
so_chb = fi(zeros(1, 2), 1, DW, 0, fm);
so_cha(:) = si_cha + si_chb;
so_chb(:) = si_cha - si_chb;
end

== matlab function r23_512p_fft/FFT_TOP/calc_unit6/bwr_unit ==
  data: si_cha input; so_cha output; so_chb output; si_chb input
function [so_cha, so_chb] = bwr_unit(si_cha, si_chb)
%BWR_UNIT Twiddle multiply after the butterfly: W^0, W^128.

DW = 13;
fm = fimath('RoundingMethod', 'Nearest', 'OverflowAction', 'Saturate', ...
    'ProductMode', 'FullPrecision', 'SumMode', 'FullPrecision');

so_cha = mul_one(si_cha, DW, fm);
so_chb = mul_neg_j(si_chb, DW, fm);
end

function y = mul_one(x, DW, fm)
y = fi(zeros(1, 2), 1, DW, 0, fm);
y(:) = x;
end

function y = mul_neg_j(x, DW, fm)
y = fi(zeros(1, 2), 1, DW, 0, fm);
y(1) = x(2);
y(2) = -x(1);
end

== matlab function r23_512p_fft/FFT_TOP/calc_unit6/r2_unit ==
  data: si_cha input; so_cha output; so_chb output; si_chb input
function [so_cha, so_chb] = r2_unit(si_cha, si_chb)
%R2_UNIT Radix-2 butterfly.

DW = 13;
fm = fimath('RoundingMethod', 'Nearest', 'OverflowAction', 'Saturate', ...
    'ProductMode', 'FullPrecision', 'SumMode', 'FullPrecision');

so_cha = fi(zeros(1, 2), 1, DW, 0, fm);
so_chb = fi(zeros(1, 2), 1, DW, 0, fm);
so_cha(:) = si_cha + si_chb;
so_chb(:) = si_cha - si_chb;
end

== matlab function r23_512p_fft/FFT_TOP/calc_unit7/bwr_unit ==
  data: si_cha input; so_cha output; so_chb output; si_chb input
function [so_cha, so_chb] = bwr_unit(si_cha, si_chb)
%BWR_UNIT Twiddle multiply after the butterfly: W^64, W^192.

DW = 13;
fm = fimath('RoundingMethod', 'Nearest', 'OverflowAction', 'Saturate', ...
    'ProductMode', 'FullPrecision', 'SumMode', 'FullPrecision');
W_A = coder.const([twiddle(64, 1, fm), twiddle(64, 2, fm)]);
W_B = coder.const([twiddle(192, 1, fm), twiddle(192, 2, fm)]);

so_cha = cmul(si_cha, W_A, DW, fm);
so_chb = cmul(si_chb, W_B, DW, fm);
end

function y = cmul(x, w, DW, fm)
y = fi(zeros(1, 2), 1, DW, 0, fm);
y(1) = x(1)*w(1) - x(2)*w(2);
y(2) = x(2)*w(1) + x(1)*w(2);
end

function w = twiddle(k, part, fm)
if part == 1
    w = fi(cos(2*pi*k/512), 1, 10, 8, fm);
else
    w = fi(-sin(2*pi*k/512), 1, 10, 8, fm);
end
end

== matlab function r23_512p_fft/FFT_TOP/calc_unit7/r2_unit ==
  data: si_cha input; so_cha output; so_chb output; si_chb input
function [so_cha, so_chb] = r2_unit(si_cha, si_chb)
%R2_UNIT Radix-2 butterfly.

DW = 13;
fm = fimath('RoundingMethod', 'Nearest', 'OverflowAction', 'Saturate', ...
    'ProductMode', 'FullPrecision', 'SumMode', 'FullPrecision');

so_cha = fi(zeros(1, 2), 1, DW, 0, fm);
so_chb = fi(zeros(1, 2), 1, DW, 0, fm);
so_cha(:) = si_cha + si_chb;
so_chb(:) = si_cha - si_chb;
end

== matlab function r23_512p_fft/FFT_TOP/calc_unit8/bwr_unit ==
  data: si_cha input; so_cha output; so_chb output; si_chb input
function [so_cha, so_chb] = bwr_unit(si_cha, si_chb)
%BWR_UNIT Twiddle multiply after the butterfly: W^0, W^(4k), k = 0..63.

DW = 14;
LEN = 64;
KW  = 6;
fm = fimath('RoundingMethod', 'Nearest', 'OverflowAction', 'Saturate', ...
    'ProductMode', 'FullPrecision', 'SumMode', 'FullPrecision');
fc = fimath('RoundingMethod', 'Floor', 'OverflowAction', 'Wrap', ...
    'ProductMode', 'FullPrecision', 'SumMode', 'FullPrecision');
ROM_B_RE = coder.const(twiddle((0:LEN-1).' * 4, 1, fm));
ROM_B_IM = coder.const(twiddle((0:LEN-1).' * 4, 2, fm));

persistent k
if isempty(k)
    k = fi(LEN - 1, 0, KW, 0, fc);
end
if k == LEN - 1
    k(:) = 0;
else
    k(:) = k + 1;
end

so_cha = mul_one(si_cha, DW, fm);
so_chb = cmul(si_chb, [ROM_B_RE(k + 1), ROM_B_IM(k + 1)], DW, fm);
end

function y = mul_one(x, DW, fm)
y = fi(zeros(1, 2), 1, DW, 0, fm);
y(:) = x;
end

function y = cmul(x, w, DW, fm)
y = fi(zeros(1, 2), 1, DW, 0, fm);
y(1) = x(1)*w(1) - x(2)*w(2);
y(2) = x(2)*w(1) + x(1)*w(2);
end

function w = twiddle(k, part, fm)
if part == 1
    w = fi(cos(2*pi*k/512), 1, 10, 8, fm);
else
    w = fi(-sin(2*pi*k/512), 1, 10, 8, fm);
end
end

== matlab function r23_512p_fft/FFT_TOP/calc_unit8/r2_unit ==
  data: si_cha input; so_cha output; so_chb output; si_chb input
function [so_cha, so_chb] = r2_unit(si_cha, si_chb)
%R2_UNIT Radix-2 butterfly.

DW = 14;
fm = fimath('RoundingMethod', 'Nearest', 'OverflowAction', 'Saturate', ...
    'ProductMode', 'FullPrecision', 'SumMode', 'FullPrecision');

so_cha = fi(zeros(1, 2), 1, DW, 0, fm);
so_chb = fi(zeros(1, 2), 1, DW, 0, fm);
so_cha(:) = si_cha + si_chb;
so_chb(:) = si_cha - si_chb;
end

== matlab function r23_512p_fft/FFT_TOP/calc_unit9/bwr_unit ==
  data: si_cha input; so_cha output; so_chb output; si_chb input
function [so_cha, so_chb] = bwr_unit(si_cha, si_chb)
%BWR_UNIT Twiddle multiply after the butterfly: W^(2k), W^(6k), k = 0..63.

DW = 14;
LEN = 64;
KW  = 6;
fm = fimath('RoundingMethod', 'Nearest', 'OverflowAction', 'Saturate', ...
    'ProductMode', 'FullPrecision', 'SumMode', 'FullPrecision');
fc = fimath('RoundingMethod', 'Floor', 'OverflowAction', 'Wrap', ...
    'ProductMode', 'FullPrecision', 'SumMode', 'FullPrecision');
ROM_A_RE = coder.const(twiddle((0:LEN-1).' * 2, 1, fm));
ROM_A_IM = coder.const(twiddle((0:LEN-1).' * 2, 2, fm));
ROM_B_RE = coder.const(twiddle((0:LEN-1).' * 6, 1, fm));
ROM_B_IM = coder.const(twiddle((0:LEN-1).' * 6, 2, fm));

persistent k
if isempty(k)
    k = fi(LEN - 1, 0, KW, 0, fc);
end
if k == LEN - 1
    k(:) = 0;
else
    k(:) = k + 1;
end

so_cha = cmul(si_cha, [ROM_A_RE(k + 1), ROM_A_IM(k + 1)], DW, fm);
so_chb = cmul(si_chb, [ROM_B_RE(k + 1), ROM_B_IM(k + 1)], DW, fm);
end

function y = cmul(x, w, DW, fm)
y = fi(zeros(1, 2), 1, DW, 0, fm);
y(1) = x(1)*w(1) - x(2)*w(2);
y(2) = x(2)*w(1) + x(1)*w(2);
end

function w = twiddle(k, part, fm)
if part == 1
    w = fi(cos(2*pi*k/512), 1, 10, 8, fm);
else
    w = fi(-sin(2*pi*k/512), 1, 10, 8, fm);
end
end

== matlab function r23_512p_fft/FFT_TOP/calc_unit9/r2_unit ==
  data: si_cha input; so_cha output; so_chb output; si_chb input
function [so_cha, so_chb] = r2_unit(si_cha, si_chb)
%R2_UNIT Radix-2 butterfly.

DW = 14;
fm = fimath('RoundingMethod', 'Nearest', 'OverflowAction', 'Saturate', ...
    'ProductMode', 'FullPrecision', 'SumMode', 'FullPrecision');

so_cha = fi(zeros(1, 2), 1, DW, 0, fm);
so_chb = fi(zeros(1, 2), 1, DW, 0, fm);
so_cha(:) = si_cha + si_chb;
so_chb(:) = si_cha - si_chb;
end

== matlab function r23_512p_fft/FFT_TOP/calc_unit15/r2_unit ==
  data: si_cha input; so_cha output; so_chb output; si_chb input
function [so_cha, so_chb] = r2_unit(si_cha, si_chb)
%R2_UNIT Radix-2 butterfly.

DW = 13;
fm = fimath('RoundingMethod', 'Nearest', 'OverflowAction', 'Saturate', ...
    'ProductMode', 'FullPrecision', 'SumMode', 'FullPrecision');

so_cha = fi(zeros(1, 2), 1, DW, 0, fm);
so_chb = fi(zeros(1, 2), 1, DW, 0, fm);
so_cha(:) = si_cha + si_chb;
so_chb(:) = si_cha - si_chb;
end

== matlab function r23_512p_fft/FFT_TOP/comm_unit00/sw_unit ==
  data: si_cha input; so_cha output; so_chb output; si_chb input
function [so_cha, so_chb] = sw_unit(si_cha, si_chb)
%SW_UNIT Commutator switch, depth 32.

N  = 32;
CW = 5;
DW = 12;
fm = fimath('RoundingMethod', 'Nearest', 'OverflowAction', 'Saturate', ...
    'ProductMode', 'FullPrecision', 'SumMode', 'FullPrecision');
fc = fimath('RoundingMethod', 'Floor', 'OverflowAction', 'Wrap', ...
    'ProductMode', 'FullPrecision', 'SumMode', 'FullPrecision');

persistent cnt sel
if isempty(cnt)
    cnt = fi(N - 1, 0, CW, 0, fc);
end
if isempty(sel)
    sel = true;
end

if cnt == N - 1
    cnt(:) = 0;
else
    cnt(:) = cnt + 1;
end
if cnt == 0
    sel = ~sel;
end

so_cha = fi(zeros(1, 2), 1, DW, 0, fm);
so_chb = fi(zeros(1, 2), 1, DW, 0, fm);
if sel
    so_cha(:) = si_chb;
    so_chb(:) = si_cha;
else
    so_cha(:) = si_cha;
    so_chb(:) = si_chb;
end
end

== matlab function r23_512p_fft/FFT_TOP/calc_unit10/r2_unit ==
  data: si_cha input; so_cha output; so_chb output; si_chb input
function [so_cha, so_chb] = r2_unit(si_cha, si_chb)
%R2_UNIT Radix-2 butterfly.

DW = 14;
fm = fimath('RoundingMethod', 'Nearest', 'OverflowAction', 'Saturate', ...
    'ProductMode', 'FullPrecision', 'SumMode', 'FullPrecision');

so_cha = fi(zeros(1, 2), 1, DW, 0, fm);
so_chb = fi(zeros(1, 2), 1, DW, 0, fm);
so_cha(:) = si_cha + si_chb;
so_chb(:) = si_cha - si_chb;
end
